simulink model "palletizing"  (R2025b)
settings: Solver=FixedStepDiscrete  StartTime=0.0  StopTime=inf  FixedStep=0.01  RelTol=1e-3
PreLoadFcn:
  | run(fullfile(fileparts(get_param(bdroot, 'FileName')), 'setupPaths.m'));
  | [rbt, robotCfg] = setupRobot();
  | robotHome = robotCfg.homeConfig;
InitFcn:
  | run(fullfile(fileparts(get_param(bdroot, 'FileName')), 'setupPaths.m'));
  | [rbt, robotCfg] = setupRobot();
  | robotHome = robotCfg.homeConfig;
undefined symbols (not defined in the file or in its folder): Actor, buildWorkCell, World
libraries: sim3dlib x2, robotsim3dlib x1
settings Model: Creator=priya  LastModifiedBy=priya

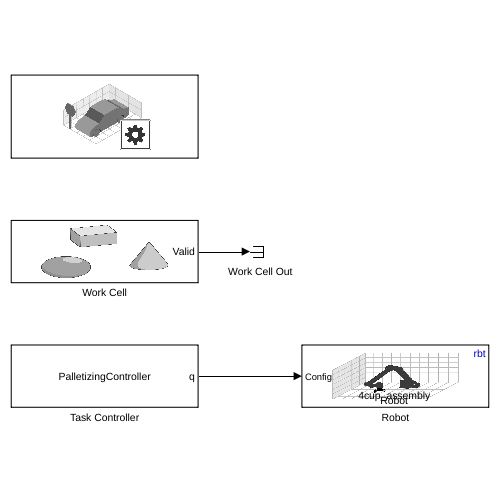
[thumbnail: Simulink's stored preview of the top-level diagram]
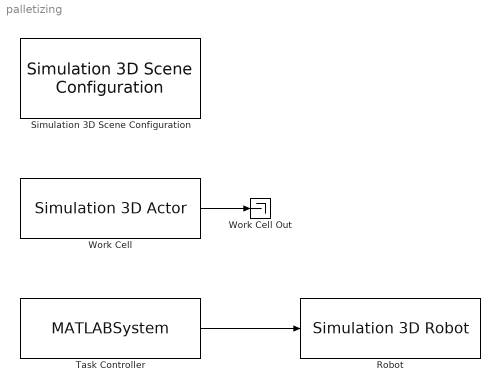
== system palletizing ==
  Robot : robotsim3dlib/Simulation 3D Robot  actorInputType=RigidBodyTree Object  RigidBodyTree=rbt  ActorName=Robot  existActorChekBox=off  initialTrans=[0 0 0]  initialRot=[0 0 0]  initialConfig=robotHome  EndEffector=4cup_assembly  eeOffsetInpChekBox=off  eeTargetTrans=[0 0 0]  eeTargetRot=[0 0 0]  enableRegionGraspChekBox=off  regionGraspInpChekBox=off  eeTargTransDiff=[0.2 0.2 0.2]  eeTargRotDiff=[0 0 0]  enableVisualVisualization=on  enableCollisionVisualization=off  collisionGeomColor=[0 1 0]  collisionGeomTransp=0.1  inpConfEnbVal=on  inpGraspEnbVal=off  inpTransEnbVal=off  outConfEnbVal=off  outGraspEnbVal=off  outTransEnbVal=off  SampleTime=0.01  ActorType=SimulinkVehicle  ID=C  aMode=6  ActorTag=Robot  Mesh=RigidBodyTree
  Simulation 3D Scene Configuration : sim3dlib/Simulation 3D Scene Configuration  Priority=0  ProjectFormat=Default Scenes  SceneDesc=Empty scene  ProjectName=/usr/local/MATLAB/R2025b/toolbox/shared/sim3d_projects/automotive_project_linux/UE/LinuxNoEditor/VehicleSimulation.sh  ScenePath=/Game/Maps/HwStrght  EnableOpenDRIVE=off  vehTagList={'<empty>';'Custom';'Scene Origin'}  vehTag=Scene Origin  AttachedCameraRelativeTranslation=[0 0 0]  FreeCameraDefaultInitialTranslation=[-6 0 2]  AttachedCameraRelativeRotation=[0 0 0]  FreeCameraDefaultInitialRotation=[0 -15 0]  ViewpointName=Custom  FreeCameraInitialTranslation=[0 0 0]  ViewpointTranslation=[0 0 0]  FreeCameraInitialRotation=[0 0 0]  ViewpointRotation=[0 0 0]  OpVisEn=off  Ts=0.02  EnableWindow=on  EnableRemoteAccess=off  EnableWeather=off  SunAzimuth=90  SunAltitude=40.0  EnableGeospatialSun=off  Latitude=0  Longitude=0  Date=2023-01-01  Time=10:30:00  GeoTimeZone=-5.0  SunDaylightSaving=off  wind=1  clouds=10  EnableVolumetricClouds=off  CloudCoverage=0  CloudAltitude=6  fog=0  rain=0  RaindropsEffect=off  SnowDensity=0  EnableGeospatial=off  TilesetSource=Earth terrain  UseTrueOrigin=off  OriginHeight=200  OriginLatitude=40.744652  OriginLongitude=-73.988864  MapStyle=Aerial  AdditionalAssetIDs=[]  UseAdvancedSunSky=off  SolarTime=11  TimeZone=-5  Day=21  Month=9  Year=2022  UseDaylightSavingTime=on  DSTStartDay=10  DSTStartMonth=3  DSTEndDay=3  DSTEndMonth=11  DSTSwitchHour=2  sensorTag=MainCamera1  sensorId=1  sensorName=MainCamera1  mountLoc=Origin  offsetFlag=off  tmountOffset=[0, 0, 0]  rmountOffset=[0, 0, 0]  HorizontalResolution=1280  VerticalResolution=720  HorizontalFOV=60  mountPoint=[0 0 0]  mountOrientation=[0 0 0]  aMode=aMode  ID=1  GeoTrigger=Inactive  ViewNameList={'Custom'}  ViewTranslationList={'[0 0 0]'}  ViewRotationList={'[0 0 0]'}
  Task Controller : MATLABSystem  System=PalletizingController  SimulateUsing=Interpreted execution
      mask Type: PalletizingController
  Work Cell : sim3dlib/Simulation 3D Actor  Priority=1  ActorName=WorkCell  ParentName=Scene Origin  Operation=Create at setup  InitScriptText=buildWorkCell(World, Actor);  SampleTime=-1  Translation=[0 0 0]  Rotation=[0 0 0]  Scale=[1 1 1]  aMode=aMode  ActorTag=WorkCell  ActorType=Sim3dActor  ID=C
  Work Cell Out : Terminator
  wires:
  Work Cell/1 -> Work Cell Out/1
  Task Controller/1 -> Robot/1
